simulink model "LKA_MIL_TestBench"  (R2026b)
settings: Solver=ode4  StopTime=SCN.StopTime  FixedStep=0.005
undefined symbols (not defined in the file): LKA, ROAD, SCN, vehicle
settings Model: Creator=rithvin007  LastModifiedBy=rithvin007
settings DebuggingCC: AlgebraicLoopMsg=error

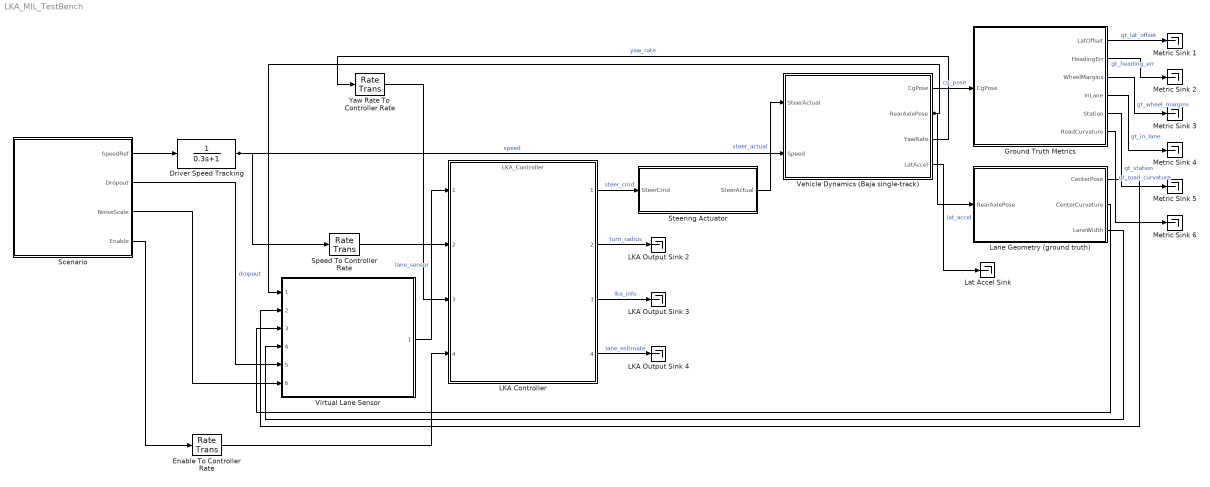
== system LKA_MIL_TestBench ==
  Driver Speed Tracking : TransferFcn  Numerator=1  Denominator=[0.3 1]
  Enable To Controller Rate : RateTransition  OutPortSampleTime=LKA.Ts
  Ground Truth Metrics : Subsystem
  LKA Controller : ModelReference  ModelNameDialog=LKA_Controller  SimulationMode=Normal  ModelReferenceVersion=1.1
  LKA Output Sink 2 : Terminator
  LKA Output Sink 3 : Terminator
  LKA Output Sink 4 : Terminator
  Lane Geometry (ground truth) : Subsystem
  Lat Accel Sink : Terminator
  Metric Sink {1..6} (6 alike) : Terminator
  Scenario : Subsystem
  Speed To Controller Rate : RateTransition  OutPortSampleTime=LKA.Ts
  Steering Actuator : Subsystem
  Vehicle Dynamics (Baja single-track) : Subsystem
  Virtual Lane Sensor : Subsystem  ReferencedSubsystem=VirtualLaneSensor
  Yaw Rate To Controller Rate : RateTransition  OutPortSampleTime=LKA.Ts
  wires:
  Lane Geometry (ground truth)/3(LaneWidth) -> Virtual Lane Sensor/4
  Lane Geometry (ground truth)/2(CenterCurvature) -> Virtual Lane Sensor/3
  Lane Geometry (ground truth)/1(CenterPose) -> Virtual Lane Sensor/2
  Ground Truth Metrics/5(Station) -> Metric Sink 5/1  "gt_station"
  Ground Truth Metrics/4(InLane) -> Metric Sink 4/1  "gt_in_lane"
  Ground Truth Metrics/3(WheelMargins) -> Metric Sink 3/1  "gt_wheel_margins"
  Ground Truth Metrics/2(HeadingErr) -> Metric Sink 2/1  "gt_heading_err"
  Ground Truth Metrics/1(LatOffset) -> Metric Sink 1/1  "gt_lat_offset"
  Vehicle Dynamics (Baja single-track)/3(YawRate) -> Yaw Rate To Controller Rate/1  "yaw_rate"
  Ground Truth Metrics/6(RoadCurvature) -> Metric Sink 6/1  "gt_road_curvature"
  Vehicle Dynamics (Baja single-track)/2(RearAxlePose) -> Lane Geometry (ground truth)/1(RearAxlePose), Virtual Lane Sensor/1
  Scenario/2(Dropout) -> Virtual Lane Sensor/5  "dropout"
  Vehicle Dynamics (Baja single-track)/4(LatAccel) -> Lat Accel Sink/1  "lat_accel"
  LKA Controller/3 -> LKA Output Sink 3/1  "lka_info"
  Steering Actuator/1(SteerActual) -> Vehicle Dynamics (Baja single-track)/1(SteerActual)  "steer_actual"
  Driver Speed Tracking/1 -> Speed To Controller Rate/1, Vehicle Dynamics (Baja single-track)/2(Speed)  "speed"
  Scenario/3(NoiseScale) -> Virtual Lane Sensor/6
  Enable To Controller Rate/1 -> LKA Controller/4
  Virtual Lane Sensor/1 -> LKA Controller/1  "lane_sensor"
  Scenario/1(SpeedRef) -> Driver Speed Tracking/1
  Scenario/4(Enable) -> Enable To Controller Rate/1
  Yaw Rate To Controller Rate/1 -> LKA Controller/3
  LKA Controller/1 -> Steering Actuator/1(SteerCmd)  "steer_cmd"
  Speed To Controller Rate/1 -> LKA Controller/2
  Vehicle Dynamics (Baja single-track)/1(CgPose) -> Ground Truth Metrics/1(CgPose)  "cg_pose"
  LKA Controller/2 -> LKA Output Sink 2/1  "turn_radius"
  LKA Controller/4 -> LKA Output Sink 4/1  "lane_estimate"

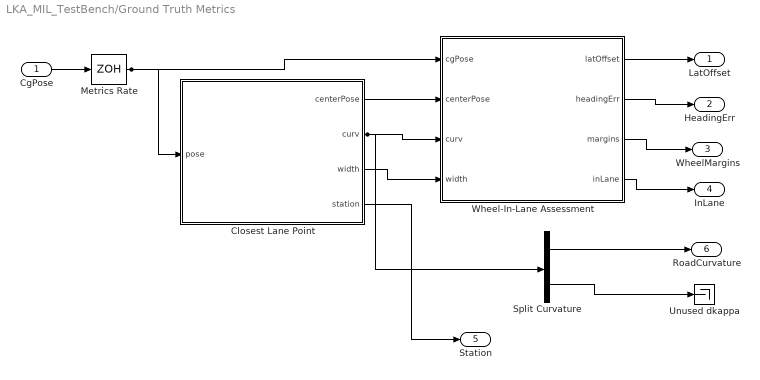
== system LKA_MIL_TestBench/Ground Truth Metrics ==
  CgPose : Inport
  Closest Lane Point : MATLAB Function  TreatAsAtomicUnit=on
  Metrics Rate : ZeroOrderHold  SampleTime=0.01
  Split Curvature : Demux  Outputs=2
  Unused dkappa : Terminator
  Wheel-In-Lane Assessment : MATLAB Function  TreatAsAtomicUnit=on
  LatOffset : Outport
  HeadingErr : Outport  Port=2
  WheelMargins : Outport  Port=3
  InLane : Outport  Port=4
  Station : Outport  Port=5
  RoadCurvature : Outport  Port=6
  wires:
  Wheel-In-Lane Assessment/4(inLane) -> InLane/1
  Wheel-In-Lane Assessment/3(margins) -> WheelMargins/1
  Wheel-In-Lane Assessment/2(headingErr) -> HeadingErr/1
  Split Curvature/1 -> RoadCurvature/1
  Closest Lane Point/4(station) -> Station/1
  Closest Lane Point/3(width) -> Wheel-In-Lane Assessment/4(width)
  Closest Lane Point/2(curv) -> Split Curvature/1, Wheel-In-Lane Assessment/3(curv)
  Wheel-In-Lane Assessment/1(latOffset) -> LatOffset/1
  Closest Lane Point/1(centerPose) -> Wheel-In-Lane Assessment/2(centerPose)
  Split Curvature/2 -> Unused dkappa/1
  Metrics Rate/1 -> Closest Lane Point/1(pose), Wheel-In-Lane Assessment/1(cgPose)
  CgPose/1 -> Metrics Rate/1

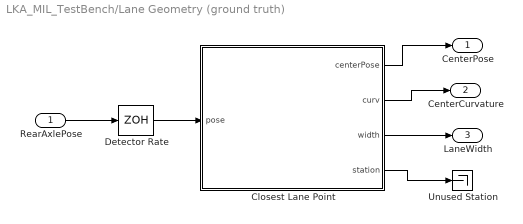
== system LKA_MIL_TestBench/Lane Geometry (ground truth) ==
  RearAxlePose : Inport
  Closest Lane Point : MATLAB Function  TreatAsAtomicUnit=on
  Detector Rate : ZeroOrderHold  SampleTime=LKA.Sen.Ts
  Unused Station : Terminator
  CenterPose : Outport
  CenterCurvature : Outport  Port=2
  LaneWidth : Outport  Port=3
  wires:
  Closest Lane Point/4(station) -> Unused Station/1
  Closest Lane Point/3(width) -> LaneWidth/1
  Closest Lane Point/2(curv) -> CenterCurvature/1
  Closest Lane Point/1(centerPose) -> CenterPose/1
  Detector Rate/1 -> Closest Lane Point/1(pose)
  RearAxlePose/1 -> Detector Rate/1

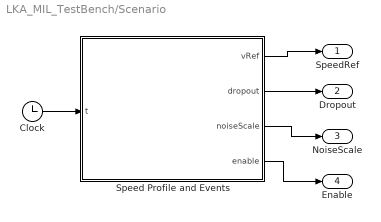
== system LKA_MIL_TestBench/Scenario ==
  Clock : Clock
  Speed Profile and Events : MATLAB Function  TreatAsAtomicUnit=on
  SpeedRef : Outport
  Dropout : Outport  Port=2
  NoiseScale : Outport  Port=3
  Enable : Outport  Port=4
  wires:
  Speed Profile and Events/4(enable) -> Enable/1
  Speed Profile and Events/3(noiseScale) -> NoiseScale/1
  Speed Profile and Events/2(dropout) -> Dropout/1
  Speed Profile and Events/1(vRef) -> SpeedRef/1
  Clock/1 -> Speed Profile and Events/1(t)

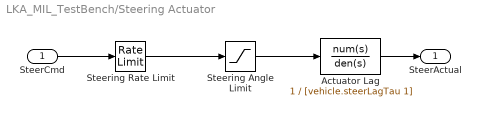
== system LKA_MIL_TestBench/Steering Actuator ==
  SteerCmd : Inport
  Actuator Lag : TransferFcn  Numerator=1  Denominator=[vehicle.steerLagTau 1]
  Steering Angle Limit : Saturate  UpperLimit=vehicle.maxSteerAngle  LowerLimit=-vehicle.maxSteerAngle
  Steering Rate Limit : RateLimiter  RisingSlewLimit=vehicle.maxSteerRate  FallingSlewLimit=-vehicle.maxSteerRate  SampleTimeMode=inherited
  SteerActual : Outport
  wires:
  Actuator Lag/1 -> SteerActual/1
  Steering Angle Limit/1 -> Actuator Lag/1
  Steering Rate Limit/1 -> Steering Angle Limit/1
  SteerCmd/1 -> Steering Rate Limit/1

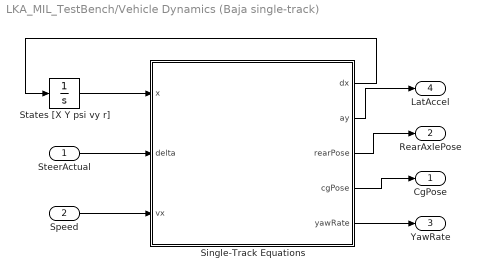
== system LKA_MIL_TestBench/Vehicle Dynamics (Baja single-track) ==
  SteerActual : Inport
  Speed : Inport  Port=2
  Single-Track Equations : MATLAB Function  TreatAsAtomicUnit=on
  States [X Y psi vy r] : Integrator  InitialCondition=SCN.X0
  CgPose : Outport
  RearAxlePose : Outport  Port=2
  YawRate : Outport  Port=3
  LatAccel : Outport  Port=4
  wires:
  Single-Track Equations/4(cgPose) -> CgPose/1
  Single-Track Equations/3(rearPose) -> RearAxlePose/1
  Single-Track Equations/5(yawRate) -> YawRate/1
  Single-Track Equations/2(ay) -> LatAccel/1
  Single-Track Equations/1(dx) -> States [X Y psi vy r]/1
  Speed/1 -> Single-Track Equations/3(vx)
  SteerActual/1 -> Single-Track Equations/2(delta)
  States [X Y psi vy r]/1 -> Single-Track Equations/1(x)

== matlab function LKA_MIL_TestBench/Vehicle Dynamics (Baja single-track)/Single-Track Equations ==
  data: x input; dx output; delta input; vx input; ay output; rearPose output; cgPose output; yawRate output; vehicle parameter
function [dx, ay, rearPose, cgPose, yawRate] = fcn(x, delta, vx, vehicle)
% Nonlinear bicycle model with saturating tyres (see lka_single_track_dynamics.m)
[dx, ay, rearPose] = lka_single_track_dynamics(x, delta, vx, vehicle);
cgPose = [x(1) x(2) x(3)];
yawRate = x(5);

== matlab function LKA_MIL_TestBench/Scenario/Speed Profile and Events ==
  data: t input; vRef output; dropout output; noiseScale output; enable output; SCN parameter
function [vRef, dropout, noiseScale, enable] = fcn(t, SCN)
% Driver speed profile v = min(V0 + a*t, VSet) and forced detector outages
vRef = min(SCN.V0 + SCN.Accel*t, SCN.VSet);
dropout = [0; 0];
for k = 1:size(SCN.Dropouts, 1)
    if t >= SCN.Dropouts(k,1) && t < SCN.Dropouts(k,2)
        side = SCN.Dropouts(k,3);
        if side == 1 || side == 3, dropout(1) = 1; end
        if side == 2 || side == 3, dropout(2) = 1; end
    end
end
noiseScale = SCN.NoiseScale;
enable = true;

== matlab function LKA_MIL_TestBench/Lane Geometry (ground truth)/Closest Lane Point ==
  data: pose input; centerPose output; curv output; width output; station output; ROAD parameter
function [centerPose, curv, width, station] = fcn(pose, ROAD)
% Foot point of the pose on the true lane centreline (windowed search, see lka_road_closest_point.m)
persistent idx
if isempty(idx), idx = 0; end
[centerPose, curv, width, station, idx] = lka_road_closest_point(pose(1), pose(2), idx, ...
    ROAD.s, ROAD.x, ROAD.y, ROAD.psi, ROAD.kappa, ROAD.dkappa, ROAD.width);

== matlab function LKA_MIL_TestBench/Ground Truth Metrics/Closest Lane Point ==
  data: pose input; centerPose output; curv output; width output; station output; ROAD parameter
function [centerPose, curv, width, station] = fcn(pose, ROAD)
% Foot point of the pose on the true lane centreline (windowed search, see lka_road_closest_point.m)
persistent idx
if isempty(idx), idx = 0; end
[centerPose, curv, width, station, idx] = lka_road_closest_point(pose(1), pose(2), idx, ...
    ROAD.s, ROAD.x, ROAD.y, ROAD.psi, ROAD.kappa, ROAD.dkappa, ROAD.width);

== matlab function LKA_MIL_TestBench/Ground Truth Metrics/Wheel-In-Lane Assessment ==
  data: cgPose input; latOffset output; centerPose input; curv input; width input; headingErr output; margins output; inLane output; ROAD parameter; vehicle parameter
function [latOffset, headingErr, margins, inLane] = fcn(cgPose, centerPose, curv, width, ROAD, vehicle)
% True CG offset, heading error and tyre-edge-to-line margins (rulebook K.2.4)
[latOffset, headingErr, margins, inLane] = lka_ground_truth_metrics(cgPose, centerPose, curv, width, ROAD.lineWidth, vehicle);
